simulink model "untitled2"  (R2023b)
settings: Solver=VariableStepAuto  StartTime=0.0  StopTime=10  MaxStep=0.0001  RelTol=1e-3
libraries: dspfdesign x1
settings Model: Creator=B03-402  LastModifiedBy=B03-402

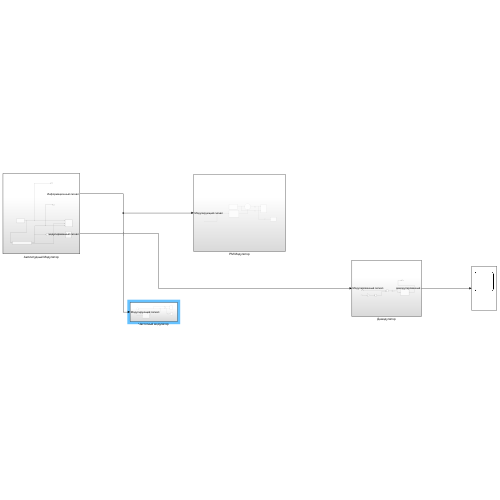
[thumbnail: Simulink's stored preview of the top-level diagram]
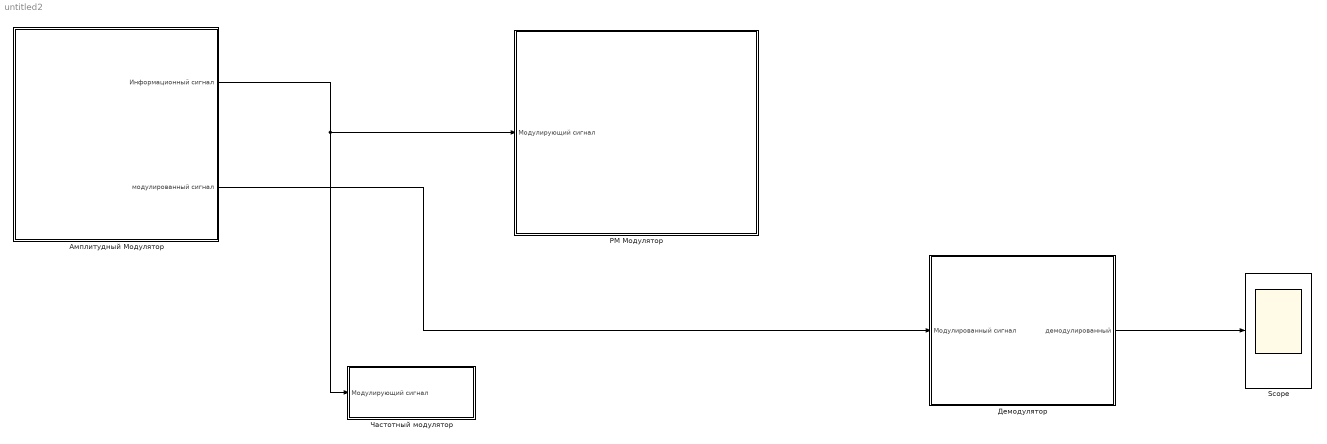
== system untitled2 ==
  PM Модулятор : Subsystem
  Scope : Scope
  Амплитудный Модулятор : Subsystem
  Демодулятор : Subsystem
  Частотный модулятор : Subsystem
  wires:
  Амплитудный Модулятор/1(Информационный сигнал) -> PM Модулятор/1(Модулирующий сигнал), Частотный модулятор/1(Модулирующий сигнал)
  Демодулятор/1(демодулированный) -> Scope/1
  Амплитудный Модулятор/2(модулированный сигнал) -> Демодулятор/1(Модулированный сигнал)

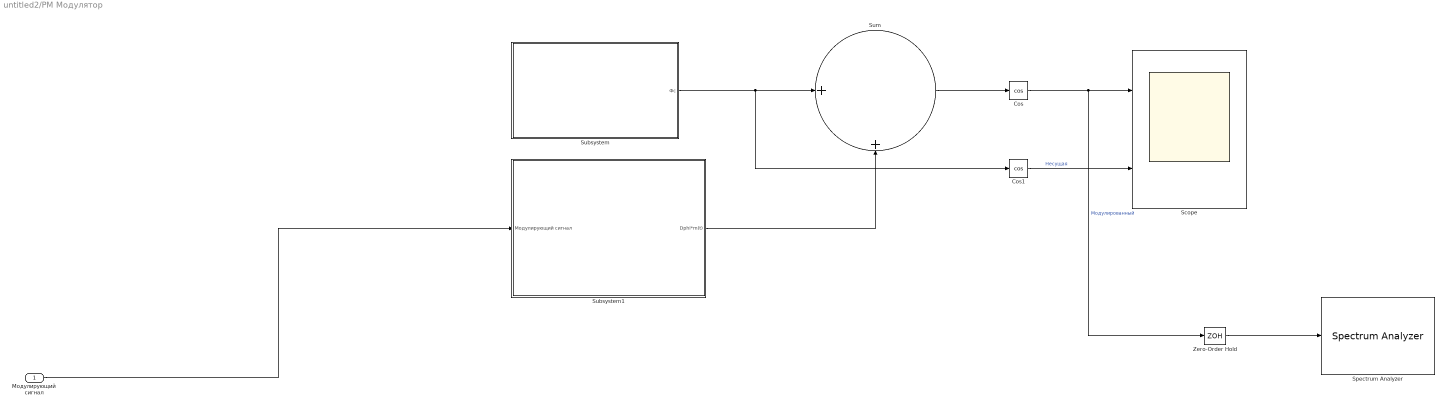
== system untitled2/PM Модулятор ==
  Модулирующий сигнал : Inport
  Cos : Trigonometry  Operator=cos
  Cos1 : Trigonometry  Operator=cos
  Scope : Scope  NumInputPorts=2
  Spectrum Analyzer : SpectrumAnalyzer  WindowPosition=[560.000000,350.000000,800.000000,500.000000,]  ScopeFrameLocation=window  YLimits=[-53.50714058,27.43298207]
  Subsystem : Subsystem  mask{Fc=300}
      mask prompts: Fc "частота несущей, гц"
  Subsystem1 : Subsystem  mask{Dphi=0.5}
  Sum : Sum  Inputs=|++
  Zero-Order Hold : ZeroOrderHold  SampleTime=1e-3
  wires:
  Subsystem/1(Фс) -> Cos1/1, Sum/1
  Модулирующий сигнал/1 -> Subsystem1/1(Модулирующий сигнал)
  Cos/1 -> Zero-Order Hold/1, Scope/1  "Модулированный"
  Cos1/1 -> Scope/2  "Несущая"
  Sum/1 -> Cos/1
  Subsystem1/1(Dphi*m(t)) -> Sum/2
  Zero-Order Hold/1 -> Spectrum Analyzer/1

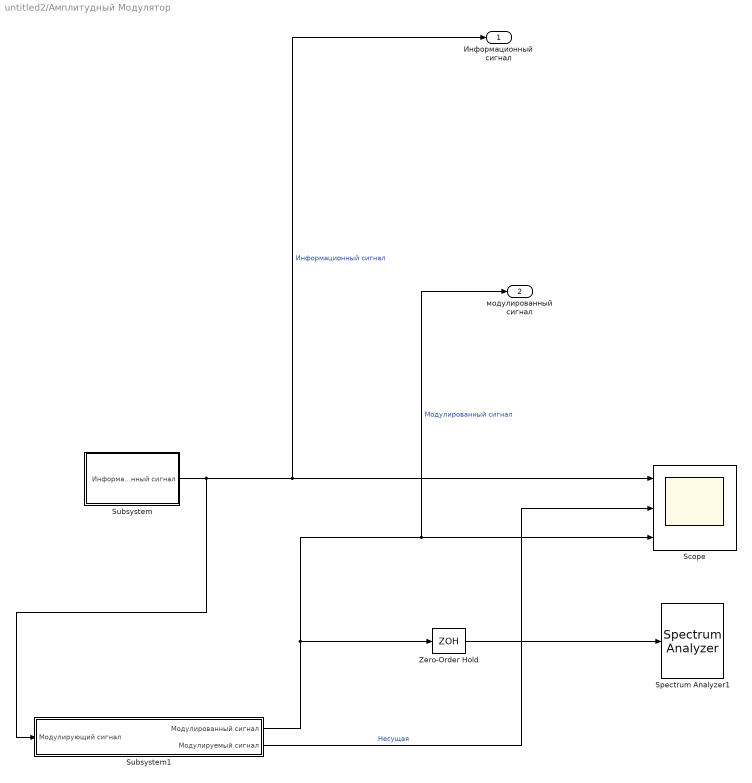
== system untitled2/Амплитудный Модулятор ==
  Scope : Scope  NumInputPorts=3
  Spectrum Analyzer1 : SpectrumAnalyzer  WindowPosition=[1.000000,41.000000,1920.000000,1137.000000,]  Visible=on  ScopeFrameLocation=window  YLimits=[-57.65717286,28.04584]
  Subsystem : Subsystem  mask{F1=40, F2=60, F3=80, F4=100}
      mask prompts: F1 "Частота1, Гц"; F2 "Частота1, Гц"; F3 "Частота3, Гц"; F4 "Частота4, Гц"
      mask DialogControl asdfsfdg Prompt: Parameters
  Subsystem1 : Subsystem  mask{Fc=300, mu=0.5}
      mask prompts: Fc "Частота несущей, Гц"; mu "Порядок модуляции mu"
  Zero-Order Hold : ZeroOrderHold  SampleTime=1e-3
  Информационный сигнал : Outport
  модулированный сигнал : Outport  Port=2
  wires:
  Subsystem/1(Информационный сигнал) -> Subsystem1/1(Модулирующий сигнал), Информационный сигнал/1, Scope/1  "Информационный сигнал"
  Subsystem1/1(Модулированный сигнал) -> Zero-Order Hold/1, модулированный сигнал/1, Scope/3  "Модулированный сигнал"
  Subsystem1/2(Модулируемый сигнал) -> Scope/2  "Несущая"
  Zero-Order Hold/1 -> Spectrum Analyzer1/1

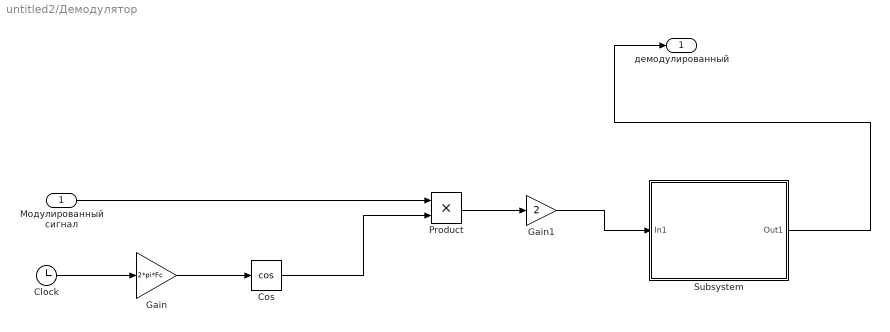
== system untitled2/Демодулятор ==
  Модулированный сигнал : Inport
  Clock : Clock
  Cos : Trigonometry  Operator=cos
  Gain : Gain  Gain=2*pi*Fc  mask{Fc=300}
      mask prompts: Fc "Частота несущей, гц"
  Gain1 : Gain  Gain=2
  Product : Product
  Subsystem : Subsystem  mask{mu=0.5, Fc=300}
      mask prompts: mu "Параметр демодулятора"; Fc "Несущая, Гц"
  демодулированный : Outport
  wires:
  Clock/1 -> Gain/1
  Gain/1 -> Cos/1
  Модулированный сигнал/1 -> Product/1
  Cos/1 -> Product/2
  Product/1 -> Gain1/1
  Gain1/1 -> Subsystem/1(In1)
  Subsystem/1(Out1) -> демодулированный/1

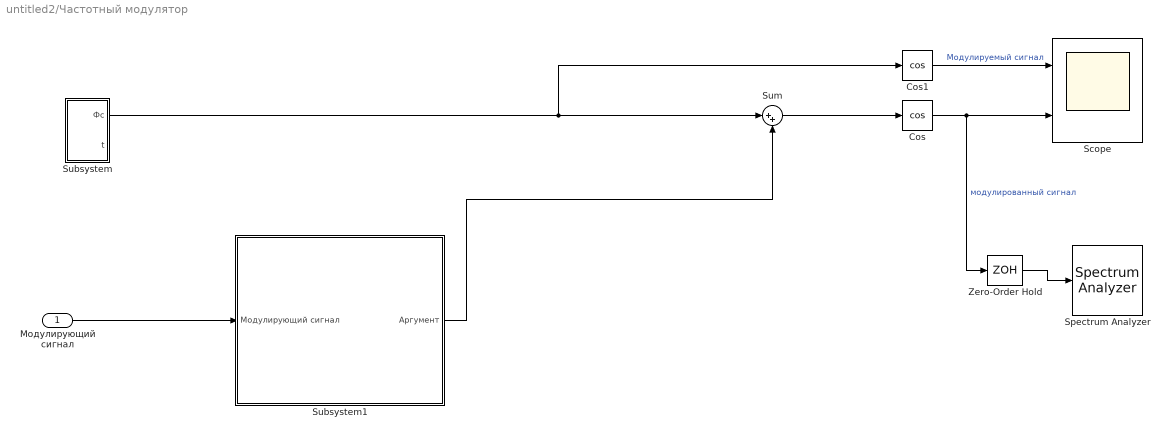
== system untitled2/Частотный модулятор ==
  Модулирующий сигнал : Inport
  Cos : Trigonometry  Operator=cos
  Cos1 : Trigonometry  Operator=cos
  Scope : Scope  NumInputPorts=2
  Spectrum Analyzer : SpectrumAnalyzer  WindowPosition=[1.000000,41.000000,1920.000000,1137.000000,]  ScopeFrameLocation=window  YLimits=[-70.50305409,28.3619246]
  Subsystem : Subsystem  mask{Fc=300}
      mask prompts: Fc "Частота несущей"
  Subsystem1 : Subsystem  mask{Df=80}
      mask prompts: Df "Девиация частоты, Гц"
  Sum : Sum  Inputs=|++
  Zero-Order Hold : ZeroOrderHold  SampleTime=1e-3
  wires:
  Модулирующий сигнал/1 -> Subsystem1/1(Модулирующий сигнал)
  Subsystem/1(Фс) -> Cos1/1, Sum/1
  Subsystem1/1(Аргумент) -> Sum/2
  Sum/1 -> Cos/1
  Cos/1 -> Zero-Order Hold/1, Scope/2  "модулированный сигнал"
  Cos1/1 -> Scope/1  "Модулируемый сигнал"
  Zero-Order Hold/1 -> Spectrum Analyzer/1

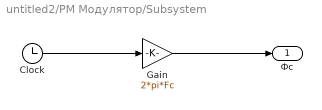
== system untitled2/PM Модулятор/Subsystem ==
  Clock : Clock
  Gain : Gain  Gain=2*pi*Fc
  Фс : Outport
  wires:
  Gain/1 -> Фс/1
  Clock/1 -> Gain/1

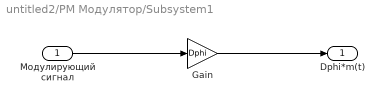
== system untitled2/PM Модулятор/Subsystem1 ==
  Модулирующий сигнал : Inport
  Gain : Gain  Gain=Dphi
  Dphi*m(t) : Outport
  wires:
  Gain/1 -> Dphi*m(t)/1
  Модулирующий сигнал/1 -> Gain/1

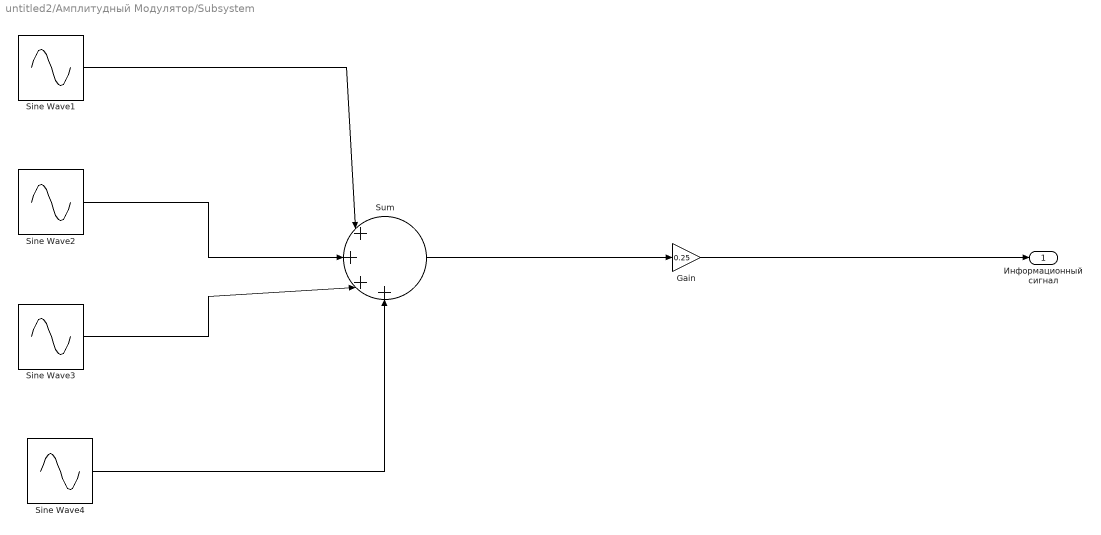
== system untitled2/Амплитудный Модулятор/Subsystem ==
  Gain : Gain  Gain=0.25
  Sine Wave1 : Sin  Frequency=2*pi*F1  SampleTime=0
  Sine Wave2 : Sin  Frequency=2*pi*F2  SampleTime=0
  Sine Wave3 : Sin  Frequency=2*pi*F3  SampleTime=0
  Sine Wave4 : Sin  Frequency=2*pi*F4  SampleTime=0
  Sum : Sum  Inputs=|++++
  Информационный сигнал : Outport
  wires:
  Sine Wave1/1 -> Sum/1
  Sine Wave2/1 -> Sum/2
  Sine Wave3/1 -> Sum/3
  Sum/1 -> Gain/1
  Sine Wave4/1 -> Sum/4
  Gain/1 -> Информационный сигнал/1

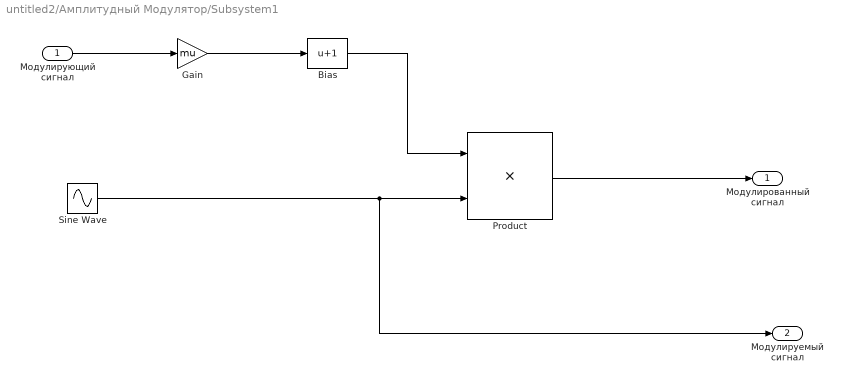
== system untitled2/Амплитудный Модулятор/Subsystem1 ==
  Модулирующий сигнал : Inport
  Bias : Bias  Bias=1  SaturateOnIntegerOverflow=off
  Gain : Gain  Gain=mu
  Product : Product
  Sine Wave : Sin  Frequency=2*pi*Fc  Phase=pi/2  SampleTime=0
  Модулированный сигнал : Outport
  Модулируемый сигнал : Outport  Port=2
  wires:
  Модулирующий сигнал/1 -> Gain/1
  Product/1 -> Модулированный сигнал/1
  Gain/1 -> Bias/1
  Sine Wave/1 -> Модулируемый сигнал/1, Product/2
  Bias/1 -> Product/1

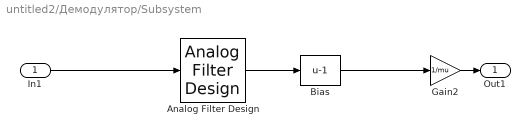
== system untitled2/Демодулятор/Subsystem ==
  In1 : Inport
  Analog Filter Design : dspfdesign/Analog Filter Design  method=Butterworth  filttype=Lowpass  N=16  Wlo=2*pi*Fc  Whi=80  Rp=2  Rs=40
  Bias : Bias  Bias=-1  SaturateOnIntegerOverflow=off
  Gain2 : Gain  Gain=1/mu
  Out1 : Outport
  wires:
  In1/1 -> Analog Filter Design/1
  Bias/1 -> Gain2/1
  Gain2/1 -> Out1/1
  Analog Filter Design/1 -> Bias/1

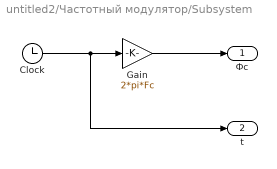
== system untitled2/Частотный модулятор/Subsystem ==
  Clock : Clock
  Gain : Gain  Gain=2*pi*Fc
  Фс : Outport
  t : Outport  Port=2
  wires:
  Clock/1 -> t/1, Gain/1
  Gain/1 -> Фс/1

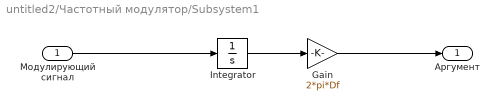
== system untitled2/Частотный модулятор/Subsystem1 ==
  Модулирующий сигнал : Inport
  Gain : Gain  Gain=2*pi*Df
  Integrator : Integrator
  Аргумент : Outport
  wires:
  Integrator/1 -> Gain/1
  Gain/1 -> Аргумент/1
  Модулирующий сигнал/1 -> Integrator/1
